simulink model "can2_mcu_odom_pack"  (R2026b)
settings: Solver=VariableStepAuto
undefined symbols (not defined in the file or in its folder): P
libraries: svdutilitieslib x1
settings Model: Creator=aomar  LastModifiedBy=aomar

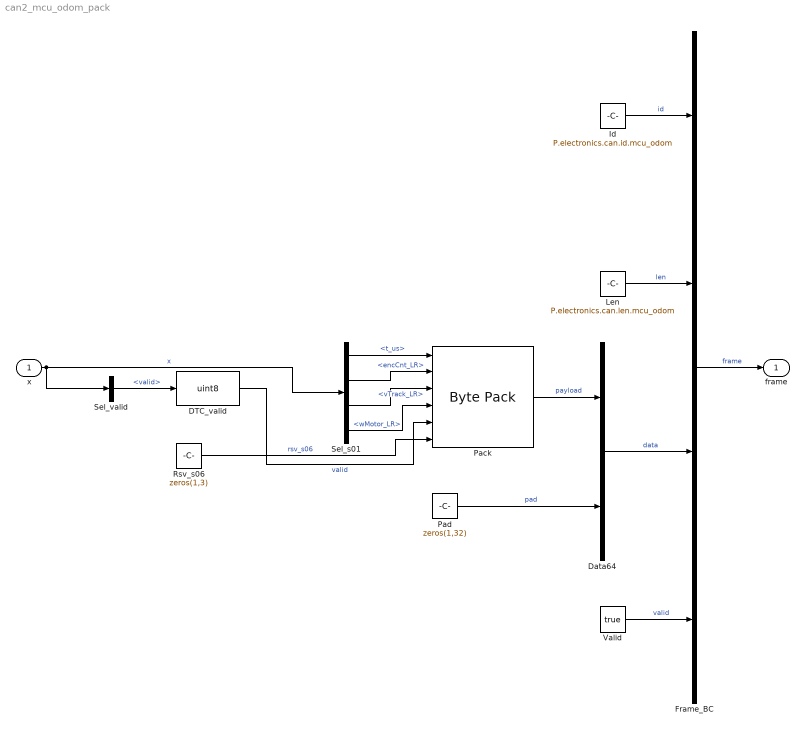
== system can2_mcu_odom_pack ==
  x : Inport  OutDataTypeStr=Bus: Bus_OdomMeas
  DTC_valid : DataTypeConversion  OutDataTypeStr=uint8  RndMeth=Round
  Data64 : Concatenate
  Frame_BC : BusCreator  Inputs=4  OutDataTypeStr=Bus: Bus_CanFrame64  NonVirtualBus=on
      settings: InheritFromInputs=off
  Id : Constant  Value=P.electronics.can.id.mcu_odom  OutDataTypeStr=uint32  SampleTime=-1
  Len : Constant  Value=P.electronics.can.len.mcu_odom  OutDataTypeStr=uint8  SampleTime=-1
  Pack : svdutilitieslib/Byte Pack  maskPackedDataType=uint8  datatypes={'uint32','int32','single','single','uint8','uint8'}  byteAlign=1  blockPlatform=arduinoert
      settings: LibrarySourceBlock=mcblib/Signal Management/Byte Pack
  Pad : Constant  Value=zeros(1,32)  OutDataTypeStr=uint8  SampleTime=-1
  Rsv_s06 : Constant  Value=zeros(1,3)  OutDataTypeStr=uint8  SampleTime=-1
  Sel_s01 : BusSelector  OutputSignals=t_us,encCnt_LR,vTrack_LR,wMotor_LR
  Sel_valid : BusSelector  OutputSignals=valid
  Valid : Constant  Value=true  OutDataTypeStr=boolean  SampleTime=-1
  frame : Outport  OutDataTypeStr=Bus: Bus_CanFrame64
  wires:
  x/1 -> Sel_s01/1, Sel_valid/1  "x"
  Sel_valid/1 -> DTC_valid/1  "<valid>"
  Rsv_s06/1 -> Pack/6  "rsv_s06"
  DTC_valid/1 -> Pack/5  "valid"
  Sel_s01/1 -> Pack/1  "<t_us>"
  Sel_s01/2 -> Pack/2  "<encCnt_LR>"
  Sel_s01/3 -> Pack/3  "<vTrack_LR>"
  Sel_s01/4 -> Pack/4  "<wMotor_LR>"
  Pad/1 -> Data64/2  "pad"
  Pack/1 -> Data64/1  "payload"
  Data64/1 -> Frame_BC/3  "data"
  Id/1 -> Frame_BC/1  "id"
  Len/1 -> Frame_BC/2  "len"
  Valid/1 -> Frame_BC/4  "valid"
  Frame_BC/1 -> frame/1  "frame"
